simulink model "PlatformDamper_Simulink_DA_Passive_MassRatio_Damping"  (R2025a)
settings: Solver=VariableStepAuto  StartTime=0  StopTime=3000  FixedStep=0.025  MaxStep=0.1  RelTol=1e-4  AbsTol=1e-6  EnableMultiTasking=on
values from neighbouring files (symbols this model uses):
  A = [O I; -M \ K -M \ C]    [Run_Active_Damping_Optimal_FullModel.m]
  A_o = [O3 I3; -M_2 \ K_2 -M_2 \ C_2]    [Run_Active_Damping_Optimal_FullModel.m]
  B = [O; M \ eye(n)]    [Run_Active_Damping_Optimal_FullModel.m]
  B_o = [O3; M_2 \ eye(3)]    [Run_Active_Damping_Optimal_FullModel.m]
  C_V = [0, 0, 0, 0, 0, 0 ... (first row only)    [Run_Active_Damping_Optimal_FullModel.m]
  C_V_o = [0 0 0; 0 -P.coes -P.coesp; 0 -P.coesp -P.coep]    [Run_Active_Damping_Optimal_FullModel.m]
  D = zeros(size(E1, 1), size(B, 2))    [Run_Active_Damping_Optimal_FullModel.m]
  D_o = zeros(3)    [Run_Active_Damping_Optimal_FullModel.m]
  E1 = [O I]    [Run_Active_Damping_Optimal_FullModel.m]
  E_o = [O3 I3]    [Run_Active_Damping_Optimal_FullModel.m]
  F_G = [0; 0; 0; 0; -P.m_TMD1 * P.g; -P.m_TMD2 * P.g]    [Run_Active_Damping_Optimal_FullModel.m]
  wc = 2 * pi * wc_hz    (= 6.28318530718)    [Run_Active_Damping_Optimal_FullModel.m]
  X2 = [0; 0; 0; 0; -static_deflection1; -static_deflection2; zeros(6, 1)]    [Run_Active_Damping_Optimal_FullModel.m]
  X2_pa = [0; 0; 0; 0; -P.m_TMD1 * P.g / P.k_pa; -P.m_TMD2 * P.g / P.k_pa1; zeros(6, 1)]    [Run_Active_Damping_Optimal_FullModel.m]
  X4 = [0; 0; 0; 0; -P.m_TMD1 * P.g / P.k_TMD1; -P.m_TMD2 * P.g / P.k_TMD2]    [Run_Active_Damping_Optimal_FullModel.m]
  X4_pa = [0; 0; 0; 0; -P.m_TMD1 * P.g / P.k_pa; -P.m_TMD2 * P.g / P.k_pa1]    [Run_Active_Damping_Optimal_FullModel.m]
  Xo_o = zeros(6, 1)    [Run_Active_Damping_Optimal_FullModel.m]
  Xo_o1 = zeros(3, 1)    [Run_Active_Damping_Optimal_FullModel.m]
undefined symbols (not defined in the file or in its folder): A_Pa
libraries: dspsrcs4 x4
Description:
  | Author: Yu Gao. Purpose: simulate uncontrolled, passive-TMD and AVD-controlled platform responses using the accompanying MATLAB driver.
settings Model: Creator=Yu Gao  LastModifiedBy=Yu Gao
settings DataIOCC: MaxDataPoints=20000
settings OptimizationCC: ExpressionDepthLimit=2147483647.0  LifeSpan=1
settings DebuggingCC: AlgebraicLoopMsg=none  UnderspecifiedInitializationDetection=Classic  MergeDetectMultiDrivingBlocksExec=none  FcnCallInpInsideContextMsg=warning  UnconnectedInputMsg=warning  UnconnectedOutputMsg=warning  UnconnectedLineMsg=warning  AllowSymbolicDim=off  StateNameClashWarn=warning  SFUnexpectedBacktrackingDiag=warning  SFNoUnconditionalDefaultTransitionDiag=warning  SFExecutionAtInitializationDiag=none  ArithmeticOperatorsInVariantConditions=warning
settings ModelReferenceCC: EnableRefExpFcnMdlSchedulingChecks=on
settings SFSimCC: SimUseLocalCustomCode=off  CustomCodeUndefinedFunction=UseInterfaceOnly
settings RTWCC: RTWUseLocalCustomCode=off  GPUComputeCapability=3.5
settings CodeAppCC: StateflowObjectComments=on
settings GRTTargetCC: TargetLangStandard=C89/C90 (ANSI)  CombineOutputUpdateFcns=off  GRTInterface=on

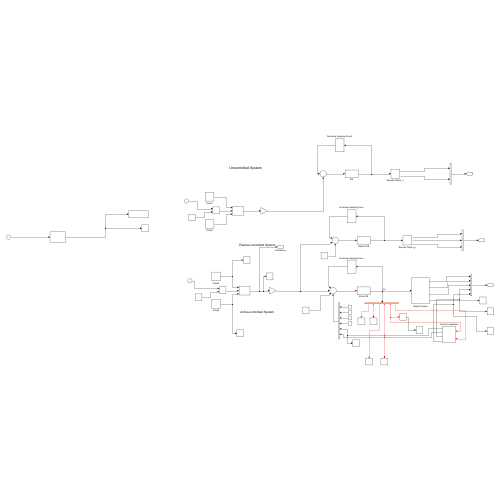
[thumbnail: Simulink's stored preview of the top-level diagram]
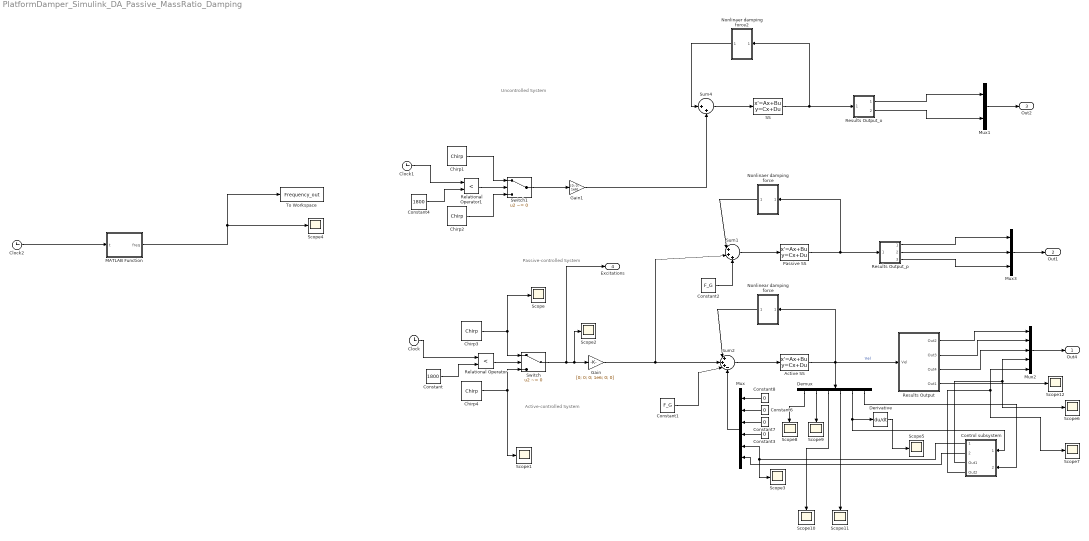
== system PlatformDamper_Simulink_DA_Passive_MassRatio_Damping ==
  note: Passive-controlled System
  note: Active-controlled System
  note: Uncontrolled System
  Active SS : StateSpace  A=A  B=B  C=E1  D=D  InitialCondition=X2  AllowTunableDMatrix=on
  Chirp1 : dspsrcs4/Chirp  sweep=Logarithmic  mode=Unidirectional  f0=0.01  f1=0.1  t1=1800  Tsweep=1800  phase=pi/2  Ts=0.025  spf=1  datatype=double  OutputFrames=off
  Chirp2 : dspsrcs4/Chirp  sweep=Logarithmic  mode=Unidirectional  f0=0.1  f1=1  t1=1200  Tsweep=1200  phase=2.2349671421856  Ts=0.025  spf=1  datatype=double  OutputFrames=off
  Chirp3 : dspsrcs4/Chirp  sweep=Logarithmic  mode=Unidirectional  f0=0.01  f1=0.1  t1=1800  Tsweep=1800  phase=pi/2  Ts=0.025  spf=1  datatype=double  OutputFrames=off
  Chirp4 : dspsrcs4/Chirp  sweep=Logarithmic  mode=Unidirectional  f0=0.1  f1=1  t1=1200  Tsweep=1200  phase=2.2349671421856  Ts=0.025  spf=1  datatype=double  OutputFrames=off
  Clock : Clock
      settings: Decimation=1800
  Clock1 : Clock
      settings: Decimation=1800
  Clock2 : Clock
  Constant : Constant  Value=1800
  Constant1 : Constant  Value=F_G
  Constant2 : Constant  Value=F_G
  Constant{3,6..8} (4 alike) : Constant  Value=0
  Constant4 : Constant  Value=1800
  Control subsystem : Subsystem
  Demux : Demux  Outputs=6
  Derivative : Derivative
  Gain : Gain  Gain=[0; 0; 0; 1e6; 0; 0]
  Gain1 : Gain  Gain=[0; 0; 1e6]
  MATLAB Function : MATLAB Function  TreatAsAtomicUnit=on
  Mux : Mux  Inputs=6
  Mux1 : Mux  Inputs=2
  Mux2 : Mux  Inputs=5
  Mux3 : Mux  Inputs=3
  Nonlinaer damping force : Subsystem
  Nonlinaer damping force2 : Subsystem
  Nonlinear damping force : Subsystem
  Passive SS : StateSpace  A=A_Pa  B=B  C=E1  D=D  InitialCondition=X2_pa  AllowTunableDMatrix=on  ContinuousStateAttributes='velocity'
  Relational Operator : RelationalOperator  Operator=<  OutDataTypeStr=boolean  RndMeth=Simplest  InputSameDT=off
  Relational Operator1 : RelationalOperator  Operator=<  OutDataTypeStr=boolean  RndMeth=Simplest  InputSameDT=off
  Results Output : Subsystem
  Results Output_o : Subsystem
  Results Output_p : Subsystem
  SS : StateSpace  A=A_o  B=B_o  C=E_o  D=D_o  InitialCondition=Xo_o  AllowTunableDMatrix=on  ContinuousStateAttributes='velocity'
  Scope{,1..12} (13 alike) : Scope
      Scope settings: ActiveDisplayYMinimum=-1  ActiveDisplayYMaximum=1
      Scope1 settings: ActiveDisplayYMinimum=-1  ActiveDisplayYMaximum=1  DataLoggingVariableName=ScopeData9
      Scope10 settings: DataLoggingVariableName=ScopeData14
      Scope11 settings: DataLoggingVariableName=ScopeData19
      Scope12 settings: DataLoggingVariableName=ScopeData20
      Scope2 settings: ActiveDisplayYMinimum=-1.3202887537832719  ActiveDisplayYMaximum=1.3047112461984907  DataLoggingVariableName=ScopeData10
      Scope3 settings: ActiveDisplayYMinimum=-1  ActiveDisplayYMaximum=1  DataLoggingVariableName=ScopeData7
      Scope4 settings: ActiveDisplayYMinimum=-870.7481848045843  ActiveDisplayYMaximum=898.46447406135087  DataLoggingVariableName=ScopeData8
      Scope5 settings: ActiveDisplayYMinimum=-0.0022359530120726785  ActiveDisplayYMaximum=0.0025518001015554597  DataLoggingVariableName=ScopeData11
      Scope6 settings: ActiveDisplayYMinimum=-0.0022359530120726785  ActiveDisplayYMaximum=0.0025518001015554597  DataLoggingVariableName=ScopeData15
      Scope7 settings: ActiveDisplayYMinimum=-0.0022359530120726785  ActiveDisplayYMaximum=0.0025518001015554597  DataLoggingVariableName=ScopeData16
      Scope8 settings: DataLoggingVariableName=ScopeData12
      Scope9 settings: DataLoggingVariableName=ScopeData13
  Sum1 : Sum  Inputs=|+++
  Sum2 : Sum  Inputs=|+++-
  Sum4 : Sum  Inputs=|++
  Switch : Switch  Criteria=u2 ~= 0  Threshold=0.5  SaturateOnIntegerOverflow=off  InputSameDT=off
  Switch1 : Switch  Criteria=u2 ~= 0  Threshold=0.5  SaturateOnIntegerOverflow=off  InputSameDT=off
  To Workspace : ToWorkspace  VariableName=Frequency_out  SaveFormat=Timeseries  SampleTime=-1
  Out4 : Outport
  Out1 : Outport  Port=2
  Out2 : Outport  Port=3
  Excitations : Outport  Port=4
  wires:
  Sum2/1 -> Active SS/1
  Active SS/1 -> Demux/1, Results Output/1(Vel), Nonlinear damping force/1(In1)  "Vel"
  Constant1/1 -> Sum2/3
  Nonlinear damping force/1(Out1) -> Sum2/1
  Results Output/2(Out3) -> Mux2/2
  Results Output/1(Out2) -> Mux2/1
  Results Output/3(Out4) -> Mux2/3
  Mux2/1 -> Out4/1
  Clock/1 -> Relational Operator/1
  Relational Operator/1 -> Switch/2
  Chirp3/1 -> Scope/1, Switch/1
  Chirp4/1 -> Scope1/1, Switch/3
  Switch/1 -> Excitations/1, Scope2/1, Gain/1
  Constant/1 -> Relational Operator/2
  Control subsystem/2(TMD2) -> Mux/6
  Constant3/1 -> Mux/4
  Constant8/1 -> Mux/1
  Constant7/1 -> Mux/3
  Constant6/1 -> Mux/2
  Mux/1 -> Sum2/4
  Control subsystem/1(TMD1) -> Mux/5, Scope3/1
  Demux/6 -> Control subsystem/2(TMD2 In)
  Clock2/1 -> MATLAB Function/1(t)
  MATLAB Function/1(freq) -> Scope4/1, To Workspace/1
  Demux/5 -> Derivative/1, Control subsystem/1(TMD1 In)
  Derivative/1 -> Scope5/1
  Control subsystem/3(Out1) -> Scope6/1, Mux2/4
  Control subsystem/4(Out2) -> Mux2/5, Scope7/1
  SS/1 -> Nonlinaer damping force2/1(In1), Results Output_o/1(In1)
  Results Output_o/1(Out1) -> Mux1/1
  Results Output_o/2(Out2) -> Mux1/2
  Nonlinaer damping force2/1(Out1) -> Sum4/1
  Mux1/1 -> Out2/1
  Sum4/1 -> SS/1
  Chirp1/1 -> Switch1/1
  Clock1/1 -> Relational Operator1/1
  Switch1/1 -> Gain1/1
  Constant4/1 -> Relational Operator1/2
  Gain1/1 -> Sum4/2
  Relational Operator1/1 -> Switch1/2
  Chirp2/1 -> Switch1/3
  Constant2/1 -> Sum1/3
  Sum1/1 -> Passive SS/1
  Gain/1 -> Sum1/2, Sum2/2
  Nonlinaer damping force/1(Out1) -> Sum1/1
  Results Output_p/3(Out3) -> Mux3/3
  Mux3/1 -> Out1/1
  Passive SS/1 -> Results Output_p/1(In1), Nonlinaer damping force/1(In1)
  Results Output_p/2(Out2) -> Mux3/2
  Results Output_p/1(Out1) -> Mux3/1
  Demux/1 -> Scope8/1
  Demux/2 -> Scope9/1
  Demux/3 -> Scope10/1
  Demux/4 -> Scope11/1
  Results Output/4(Out1) -> Scope12/1

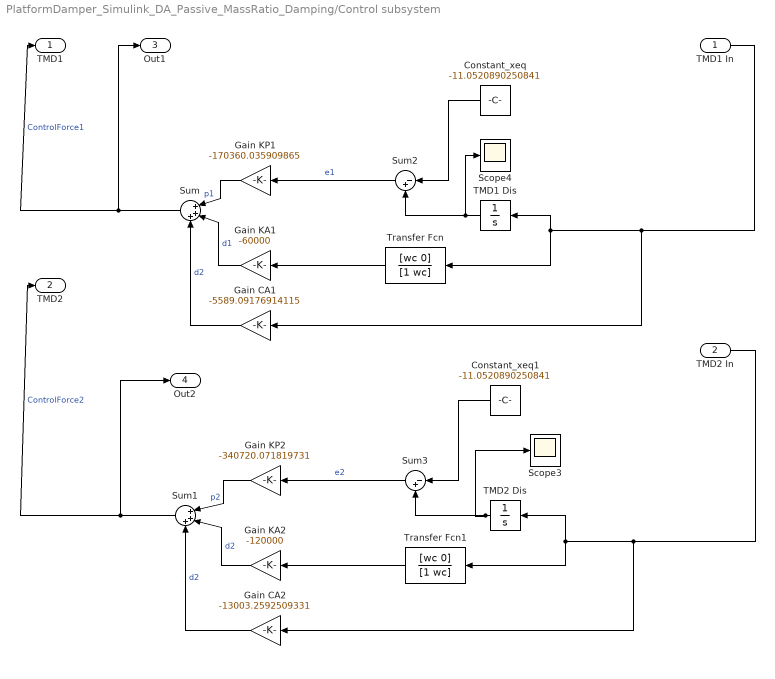
== system PlatformDamper_Simulink_DA_Passive_MassRatio_Damping/Control subsystem ==
  TMD1 In : Inport
  TMD2 In : Inport  Port=2
  Constant_xeq : Constant  Value=-11.0520890250841
  Constant_xeq1 : Constant  Value=-11.0520890250841
  Gain CA1 : Gain  Gain=-5589.09176914115
  Gain CA2 : Gain  Gain=-13003.2592509331
  Gain KA1 : Gain  Gain=-60000
  Gain KA2 : Gain  Gain=-120000
  Gain KP1 : Gain  Gain=-170360.035909865
  Gain KP2 : Gain  Gain=-340720.071819731
  Scope3 : Scope
      settings: ActiveDisplayYMinimum=-1  ActiveDisplayYMaximum=1  DataLoggingVariableName=ScopeData17
  Scope4 : Scope
      settings: ActiveDisplayYMinimum=-1  ActiveDisplayYMaximum=1  DataLoggingVariableName=ScopeData18
  Sum : Sum  Inputs=|+++
  Sum1 : Sum  Inputs=|+++
  Sum2 : Sum  Inputs=|-+
  Sum3 : Sum  Inputs=|-+
  TMD1 Dis : Integrator  InitialCondition=-11.0520890250841
  TMD2 Dis : Integrator  InitialCondition=-11.0520890250841
  Transfer Fcn : TransferFcn  Numerator=[wc 0]  Denominator=[1 wc]
  Transfer Fcn1 : TransferFcn  Numerator=[wc 0]  Denominator=[1 wc]
  TMD1 : Outport
  TMD2 : Outport  Port=2
  Out1 : Outport  Port=3
  Out2 : Outport  Port=4
  wires:
  Gain KA1/1 -> Sum/2  "d1"
  Gain KP1/1 -> Sum/1  "p1"
  TMD1 Dis/1 -> Scope4/1, Sum2/2
  Constant_xeq/1 -> Sum2/1
  Sum2/1 -> Gain KP1/1  "e1"
  Gain KP2/1 -> Sum1/1  "p2"
  Constant_xeq1/1 -> Sum3/1
  TMD2 Dis/1 -> Scope3/1, Sum3/2
  Gain KA2/1 -> Sum1/2  "d2"
  Sum3/1 -> Gain KP2/1  "e2"
  Sum1/1 -> TMD2/1, Out2/1  "ControlForce2"
  TMD2 In/1 -> Gain CA2/1, Transfer Fcn1/1, TMD2 Dis/1
  Transfer Fcn/1 -> Gain KA1/1
  Transfer Fcn1/1 -> Gain KA2/1
  Sum/1 -> TMD1/1, Out1/1  "ControlForce1"
  TMD1 In/1 -> Gain CA1/1, Transfer Fcn/1, TMD1 Dis/1
  Gain CA1/1 -> Sum/3  "d2"
  Gain CA2/1 -> Sum1/3  "d2"

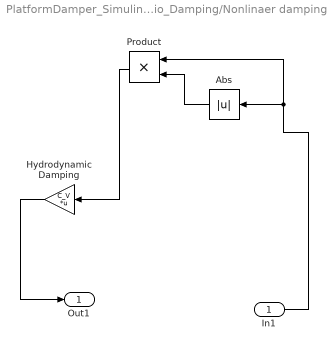
== system PlatformDamper_Simulink_DA_Passive_MassRatio_Damping/Nonlinaer damping force ==
  In1 : Inport
  Abs : Abs  SaturateOnIntegerOverflow=off
  Hydrodynamic Damping : Gain  Gain=C_V  Multiplication=Matrix(K*u)
  Product : Product
  Out1 : Outport
  wires:
  Abs/1 -> Product/2
  In1/1 -> Abs/1, Product/1
  Hydrodynamic Damping/1 -> Out1/1
  Product/1 -> Hydrodynamic Damping/1

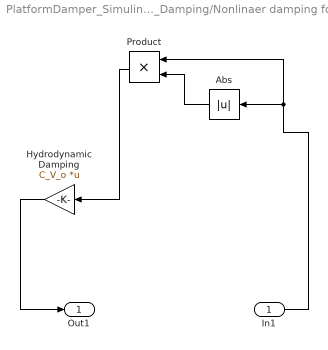
== system PlatformDamper_Simulink_DA_Passive_MassRatio_Damping/Nonlinaer damping force2 ==
  In1 : Inport
  Abs : Abs  SaturateOnIntegerOverflow=off
  Hydrodynamic Damping : Gain  Gain=C_V_o  Multiplication=Matrix(K*u)
  Product : Product
  Out1 : Outport
  wires:
  Abs/1 -> Product/2
  In1/1 -> Abs/1, Product/1
  Hydrodynamic Damping/1 -> Out1/1
  Product/1 -> Hydrodynamic Damping/1

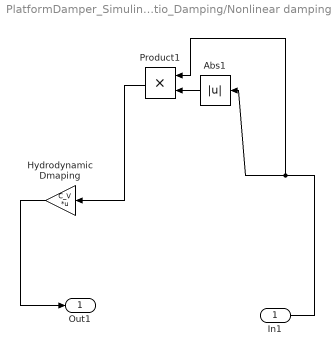
== system PlatformDamper_Simulink_DA_Passive_MassRatio_Damping/Nonlinear damping force ==
  In1 : Inport
  Abs1 : Abs  SaturateOnIntegerOverflow=off
  Hydrodynamic Dmaping : Gain  Gain=C_V  Multiplication=Matrix(K*u)
  Product1 : Product
  Out1 : Outport
  wires:
  Product1/1 -> Hydrodynamic Dmaping/1
  In1/1 -> Abs1/1, Product1/1
  Abs1/1 -> Product1/2
  Hydrodynamic Dmaping/1 -> Out1/1

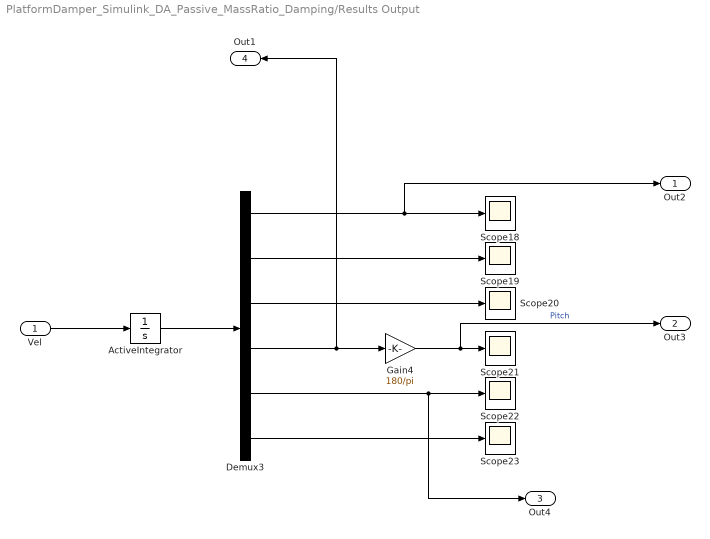
== system PlatformDamper_Simulink_DA_Passive_MassRatio_Damping/Results Output ==
  Vel : Inport
  ActiveIntegrator : Integrator  InitialCondition=X4
  Demux3 : Demux  Outputs=6
  Gain4 : Gain  Gain=180/pi
  Scope{18..23} (6 alike) : Scope
      Scope18 settings: ActiveDisplayYMinimum=-2.09733913326829  ActiveDisplayYMaximum=0.9618739340364324
      Scope19 settings: ActiveDisplayYMinimum=-1  ActiveDisplayYMaximum=1  DataLoggingVariableName=ScopeData2
      Scope20 settings: ActiveDisplayYMinimum=-1  ActiveDisplayYMaximum=1  DataLoggingVariableName=ScopeData3
      Scope21 settings: ActiveDisplayYMinimum=-25.949700094975672  ActiveDisplayYMaximum=27.832084800116874  DataLoggingVariableName=ScopeData4
      Scope22 settings: ActiveDisplayYMinimum=-1  ActiveDisplayYMaximum=1  DataLoggingVariableName=ScopeData5
      Scope23 settings: ActiveDisplayYMinimum=-1  ActiveDisplayYMaximum=1  DataLoggingVariableName=ScopeData6
  Out2 : Outport
  Out3 : Outport  Port=2
  Out4 : Outport  Port=3
  Out1 : Outport  Port=4
  wires:
  Demux3/6 -> Scope23/1
  Demux3/2 -> Scope19/1
  Demux3/5 -> Scope22/1, Out4/1
  Demux3/3 -> Scope20/1
  Vel/1 -> ActiveIntegrator/1
  Demux3/4 -> Out1/1, Gain4/1
  Demux3/1 -> Out2/1, Scope18/1
  Gain4/1 -> Out3/1, Scope21/1  "Pitch"
  ActiveIntegrator/1 -> Demux3/1

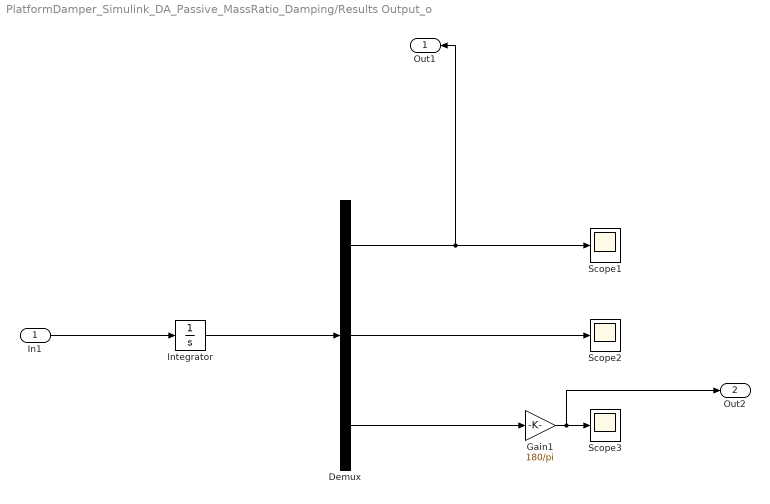
== system PlatformDamper_Simulink_DA_Passive_MassRatio_Damping/Results Output_o ==
  In1 : Inport
  Demux : Demux  Outputs=3
  Gain1 : Gain  Gain=180/pi
  Integrator : Integrator  InitialCondition=Xo_o1
  Scope1 : Scope
      settings: ActiveDisplayYMinimum=-2.2119835346158072  ActiveDisplayYMaximum=1.0001901860541524
  Scope2 : Scope
      settings: ActiveDisplayYMinimum=-0.31887  ActiveDisplayYMaximum=0.31294  DataLoggingVariableName=ScopeData2
  Scope3 : Scope
      settings: ActiveDisplayYMinimum=-11.295320510837982  ActiveDisplayYMaximum=9.8144222019721781  DataLoggingVariableName=ScopeData3
  Out1 : Outport
  Out2 : Outport  Port=2
  wires:
  In1/1 -> Integrator/1
  Demux/2 -> Scope2/1
  Demux/1 -> Out1/1, Scope1/1
  Demux/3 -> Gain1/1
  Integrator/1 -> Demux/1
  Gain1/1 -> Out2/1, Scope3/1

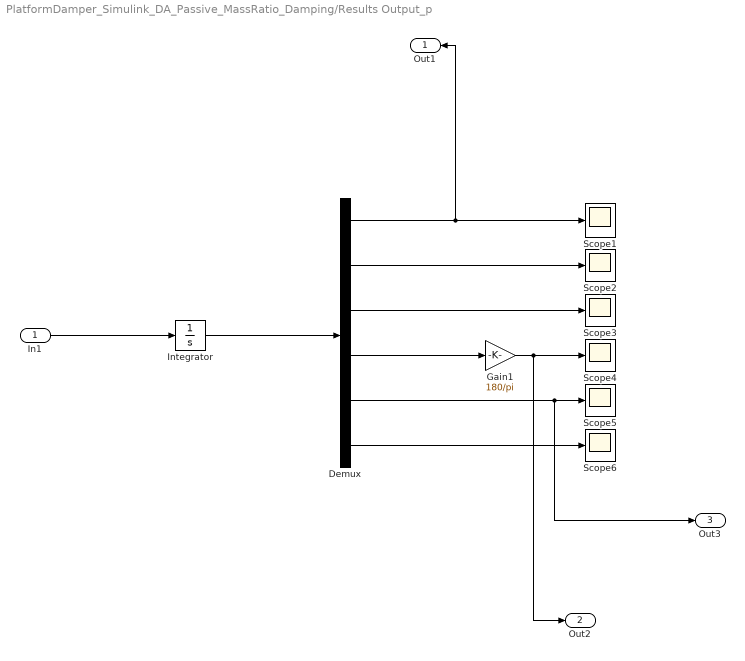
== system PlatformDamper_Simulink_DA_Passive_MassRatio_Damping/Results Output_p ==
  In1 : Inport
  Demux : Demux  Outputs=6
  Gain1 : Gain  Gain=180/pi
  Integrator : Integrator  InitialCondition=X4_pa
  Scope{1..6} (6 alike) : Scope
      Scope1 settings: ActiveDisplayYMinimum=-3.03064  ActiveDisplayYMaximum=1.27398
      Scope2 settings: ActiveDisplayYMinimum=-0.31887  ActiveDisplayYMaximum=0.31294  DataLoggingVariableName=ScopeData2
      Scope3 settings: ActiveDisplayYMinimum=-0.7220562312150498  ActiveDisplayYMaximum=0.753041052271124  DataLoggingVariableName=ScopeData3
      Scope4 settings: ActiveDisplayYMinimum=-0.99561144760772446  ActiveDisplayYMaximum=1.9592994399704016
      Scope5 settings: ActiveDisplayYMinimum=-367.37626642275569  ActiveDisplayYMaximum=19.101228803292891  DataLoggingVariableName=ScopeData5
      Scope6 settings: ActiveDisplayYMinimum=-5.57256  ActiveDisplayYMaximum=5.46245  DataLoggingVariableName=ScopeData6
  Out1 : Outport
  Out2 : Outport  Port=2
  Out3 : Outport  Port=3
  wires:
  In1/1 -> Integrator/1
  Demux/2 -> Scope2/1
  Gain1/1 -> Out2/1, Scope4/1
  Demux/5 -> Out3/1, Scope5/1
  Demux/1 -> Out1/1, Scope1/1
  Demux/4 -> Gain1/1
  Demux/3 -> Scope3/1
  Demux/6 -> Scope6/1
  Integrator/1 -> Demux/1

== matlab function PlatformDamper_Simulink_DA_Passive_MassRatio_Damping/MATLAB Function ==
  data: t input; freq output
function freq = excitation_frequency(t)
% 计算激励频率
% 输入: t - 仿真时间(s)
% 输出: freq - 瞬时频率(Hz)

% 第一段: 0-1800s, 0.01-0.1 Hz
if t <= 1800
    freq = 0.01 * (0.1/0.01)^(t/1800);
% 第二段: 1800-3000s, 0.1-1 Hz  
elseif t <= 3000
    t_local = t - 1800;
    freq = 0.1 * (1/0.1)^(t_local/1200);
else
    freq = 1;  % 保持最终频率
end

% 确保频率在合理范围内
freq = max(0.01, min(1.0, freq));
end
